simulink model "adder_tree_test"  (Simulink 7.4)
settings: Solver=VariableStepDiscrete  SolverMode=SingleTasking  StartTime=0.0  StopTime=256  RelTol=1e-3
libraries: xbsIndex_r4 x23
settings Model: Creator=User  LastModifiedBy=sgowda
settings OptimizationCC: InitFltsAndDblsToZero=on
settings DebuggingCC: SaveWithDisabledLinksMsg=none

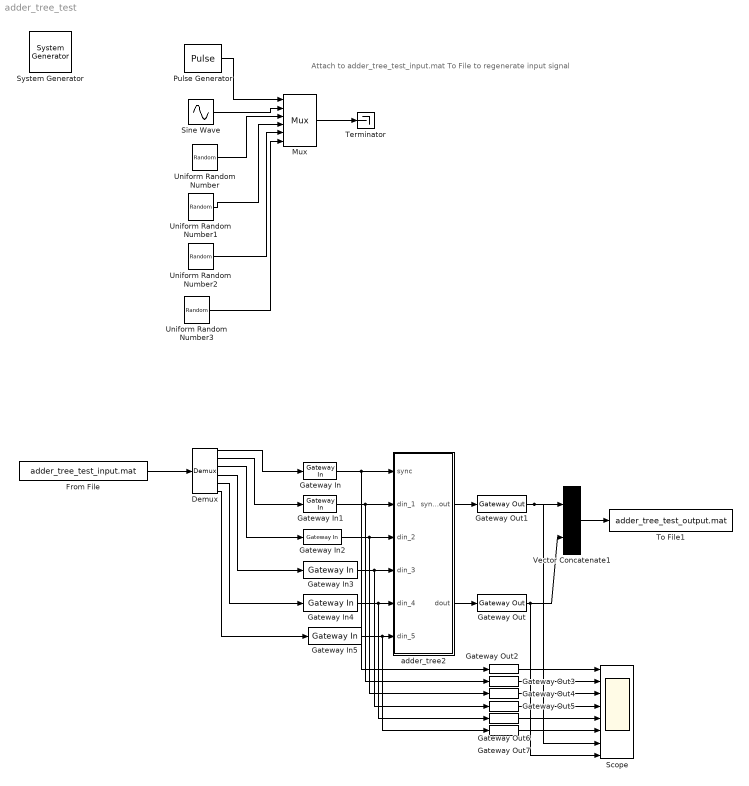
== system adder_tree_test ==
  note: Attach to adder_tree_test_input.mat To File
      | to regenerate input signal
  " System Generator" : xbsIndex_r4/ System Generator  Tag=genX  SystemSampleTime=-1  xilinxfamily=Virtex4  part=xc4vsx35  speed=-10  package=ff668  synthesis_tool=XST  clock_wrapper=Clock Enables  directory=./netlist  testbench=off  simulink_period=1  sysclk_period=10  dcm_input_clock_period=100  incr_netlist=off  trim_vbits=Everywhere in SubSystem  dbl_ovrd=According to Block Masks  core_generation=According to Block Masks  run_coregen=off  deprecated_control=off  eval_field=0  block_type=sysgen
      settings: block_version=8.2.02
  Demux : Demux  Outputs=6
  From File : FromFile  FileName=adder_tree_test_input.mat  SampleTime=1
  Gateway In : xbsIndex_r4/Gateway In  arith_type=Boolean  n_bits=25  bin_pt=0  quantization="Round  (unbiased: +/- Inf)"  overflow=Saturate  period=1  dbl_ovrd=off  timing_constraint=None  locs_specified=off  LOCs={}  hdl_port=on  block_type=gatewayin
      settings: infoedit="Gateway in block.  Converts inputs of type Simulink integer, double and fixed point to  Xilinx fixed point type.<P><P>Hardware notes:  In hardware these blocks become top level input ports."  block_version=10.1.1
  Gateway In1 : xbsIndex_r4/Gateway In  arith_type="Signed  (2's comp)"  n_bits=8  bin_pt=0  quantization=Truncate  overflow=Saturate  period=1  dbl_ovrd=off  timing_constraint=None  locs_specified=off  LOCs={}  hdl_port=on  block_type=gatewayin
      settings: infoedit="Gateway in block.  Converts inputs of type Simulink integer, double and fixed point to  Xilinx fixed point type.<P><P>Hardware notes:  In hardware these blocks become top level input ports."  block_version=10.1.1
  Gateway In{2..5} (4 alike) : xbsIndex_r4/Gateway In  arith_type="Signed  (2's comp)"  n_bits=8  bin_pt=0  quantization="Round  (unbiased: +/- Inf)"  overflow=Saturate  period=1  dbl_ovrd=off  timing_constraint=None  locs_specified=off  LOCs={}  hdl_port=on  block_type=gatewayin
      settings: infoedit="Gateway in block.  Converts inputs of type Simulink integer, double and fixed point to  Xilinx fixed point type.<P><P>Hardware notes:  In hardware these blocks become top level input ports."  block_version=10.1.1
  Gateway Out{,1..7} (8 alike) : xbsIndex_r4/Gateway Out  hdl_port=on  timing_constraint=None  locs_specified=off  LOCs={}  block_type=gatewayout
      settings: infoedit="Gateway out block.  Converts Xilinx fixed point inputs into ouputs of type Simulink integer, double, or fixed point.<P><P>Hardware notes:  In hardware these blocks become top level output ports or are discarded, depending on how they are configured."  block_version=10.1.1
  Mux : Mux  Inputs=6
  Pulse Generator : DiscretePulseGenerator  Amplitude=1  Period=32  PulseWidth=1  PhaseDelay=10  SampleTime=1
  Scope : Scope  NumInputPorts=8
      settings: TimeRange=1200  YMin=0~-200~-200~-200~0~-400~-5~-5  YMax=1~200~200~200~1~400~5~5
  Sine Wave : Sin  SineType=Sample based  Amplitude=128  Bias=0  Frequency=1  Phase=0  Samples=256  SampleTime=1  Offset=0
  Terminator : Terminator
  To File1 : ToFile  Filename=adder_tree_test_output.mat  MatrixName=output
  Uniform Random Number : UniformRandomNumber  Minimum=-128  Maximum=127  SampleTime=1
  Uniform Random Number1 : UniformRandomNumber  Minimum=-128  Maximum=127  Seed=1  SampleTime=1
  Uniform Random Number2 : UniformRandomNumber  Minimum=-128  Maximum=127  Seed=2  SampleTime=1
  Uniform Random Number3 : UniformRandomNumber  Minimum=-128  Maximum=127  Seed=3  SampleTime=1
  Vector Concatenate1 : Concatenate  Mode=Vector
  adder_tree2 : Subsystem  AncestorBlock=casper_library/Misc/adder_tree  mask(adder_tree){n_inputs=5, latency=3, quantization=Truncate, overflow=Wrap, mode=Fabric}
      mask prompts: n_inputs "Number of Inputs"; latency "Add Latency"; mode "Implementation Mode"
      mask help: Sums all inputs using a tree of adds and delays.
      mask init:
      | config.source = str2func('adder_tree_init_xblock');
      | config.toplevel = gcb;
      | xBlock(config, {n_inputs, latency, quantization, overflow, mode})
      | 
      | % adder_tree_init(gcb, ...
      | %     'n_inputs', n_inputs, ...
      | %     'latency', latency);
      settings: AttributesFormatString=latency 9
      mask Help: eval('xlWeb([getenv(''MLIB_ROOT''), ''\doc\htmlblocks\sp_adder_tree\sp_adder_tree.html''])')
      mask StyleString: edit,edit,popup(Truncate|Round (unbiased: +/- Inf)),popup(Wrap|Saturate|Flag as error),popup(DSP48e|Behavioral|Fabric)
  wires:
  Pulse Generator/1 -> Mux/1
  Gateway In/1 -> Gateway Out2/1, adder_tree2/1(sync)
  Gateway In1/1 -> Gateway Out3/1, adder_tree2/2(din_1)
  Gateway In2/1 -> Gateway Out4/1, adder_tree2/3(din_2)
  Gateway In3/1 -> Gateway Out5/1, adder_tree2/4(din_3)
  adder_tree2/1(sync_out) -> Gateway Out1/1
  adder_tree2/2(dout) -> Gateway Out/1
  Gateway Out1/1 -> Vector Concatenate1/1, Scope/7
  Gateway Out/1 -> Vector Concatenate1/2, Scope/8
  Vector Concatenate1/1 -> To File1/1
  Demux/1 -> Gateway In/1
  Demux/2 -> Gateway In1/1
  Demux/3 -> Gateway In2/1
  Demux/4 -> Gateway In3/1
  Mux/1 -> Terminator/1
  Sine Wave/1 -> Mux/2
  Gateway Out2/1 -> Scope/1
  Gateway Out3/1 -> Scope/2
  Gateway Out4/1 -> Scope/3
  Gateway Out5/1 -> Scope/4
  Uniform Random Number/1 -> Mux/3
  Uniform Random Number1/1 -> Mux/4
  Uniform Random Number2/1 -> Mux/5
  Demux/5 -> Gateway In4/1
  Gateway In4/1 -> Gateway Out6/1, adder_tree2/5(din_4)
  Uniform Random Number3/1 -> Mux/6
  Demux/6 -> Gateway In5/1
  Gateway In5/1 -> Gateway Out7/1, adder_tree2/6(din_5)
  Gateway Out6/1 -> Scope/5
  Gateway Out7/1 -> Scope/6
  From File/1 -> Demux/1

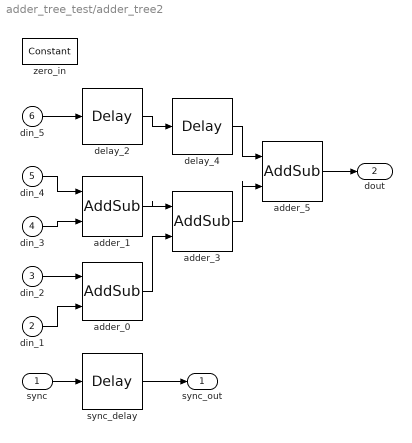
== system adder_tree_test/adder_tree2 ==
  sync : Inport  OutDataType=sfix(16)  OutScaling=2^0
  din_1 : Inport  Port=2
  din_2 : Inport  Port=3
  din_3 : Inport  Port=4
  din_4 : Inport  Port=5
  din_5 : Inport  Port=6
  adder_{0..1,3,5} (4 alike) : xbsIndex_r4/AddSub  mode=Addition  use_carryin=off  use_carryout=off  en=off  latency=3  precision=Full  arith_type=Unsigned  n_bits=16  bin_pt=14  quantization=Truncate  overflow=Wrap  dbl_ovrd=off  use_behavioral_HDL=off  hw_selection=Fabric  pipelined=off  block_type=addsub
  delay_2 : xbsIndex_r4/Delay  en=off  latency=3  dbl_ovrd=off  reg_retiming=off  block_type=delay
      settings: block_version=11.4
  delay_4 : xbsIndex_r4/Delay  en=off  latency=3  dbl_ovrd=off  reg_retiming=off  block_type=delay
      settings: block_version=11.4
  sync_delay : xbsIndex_r4/Delay  en=off  latency=9  dbl_ovrd=off  reg_retiming=off  block_type=delay
      settings: block_version=11.4
  zero_in : xbsIndex_r4/Constant  arith_type=Unsigned  const=0  n_bits=18  bin_pt=17  explicit_period=off  period=1  equ=P=C  opselect=C  inp2=PCIN>>17  opr=+  inp1=P  carry=CIN  dbl_ovrd=off  block_type=constant
      settings: block_version=11.4
  sync_out : Outport  OutDataType=sfix(16)  OutScaling=2^0
  dout : Outport  Port=2  OutDataType=sfix(16)  OutScaling=2^0
  wires:
  adder_5/1 -> dout/1
  adder_3/1 -> adder_5/2
  delay_4/1 -> adder_5/1
  delay_2/1 -> delay_4/1
  adder_0/1 -> adder_3/2
  adder_1/1 -> adder_3/1
  din_5/1 -> delay_2/1
  din_3/1 -> adder_1/2
  din_4/1 -> adder_1/1
  din_1/1 -> adder_0/2
  din_2/1 -> adder_0/1
  sync_delay/1 -> sync_out/1
  sync/1 -> sync_delay/1
